simulink model "hdlFrame_LineBufferReuse_MLFB"  (R2025a)
settings: Solver=VariableStepAuto  StartTime=0.0  StopTime=1  RelTol=1e-3
libraries: visionsources x1
settings Model: Creator=navan  LastModifiedBy=kkintali
settings SolverCC: MaxZcPerStep=1.0
settings OptimizationCC: ReuseModelBlockBuffer=off
settings DebuggingCC: UnconnectedInputMsg=warning  UnconnectedOutputMsg=warning  UnconnectedLineMsg=warning
settings ModelReferenceCC: EnableRefExpFcnMdlSchedulingChecks=on
settings SFSimCC: SimDynamicStringBufferSize=Inherit from code generation settings
settings RTWCC: GPUComputeCapability=3.5  DLArmComputeVersion=19.05

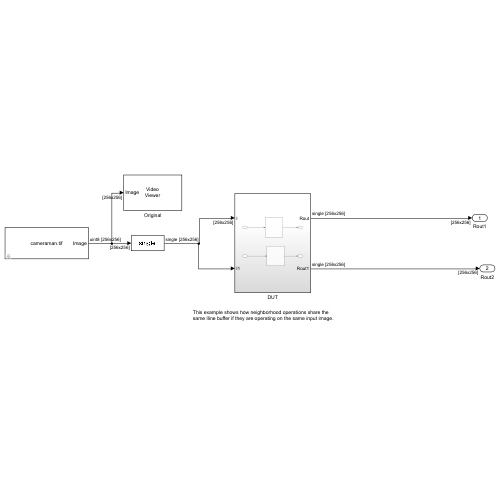
[thumbnail: Simulink's stored preview of the top-level diagram]
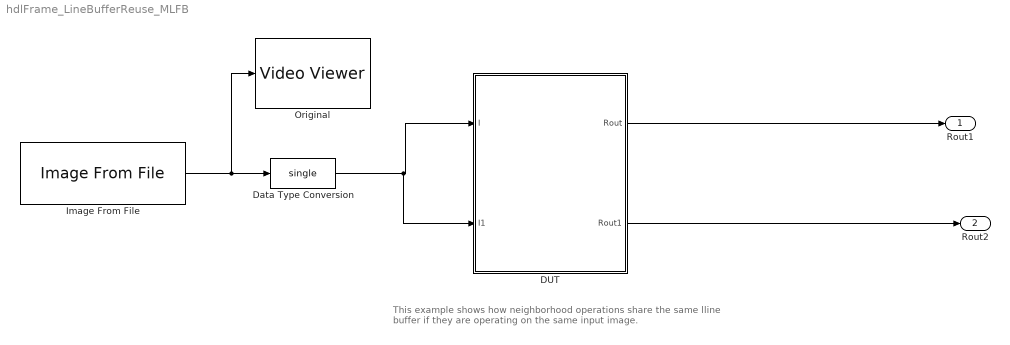
== system hdlFrame_LineBufferReuse_MLFB ==
  note: This example shows how neighborhood operations share the same lline buffer if they are operating on the same input image.
  DUT : Subsystem
  Data Type Conversion : DataTypeConversion  OutDataTypeStr=single  SaturateOnIntegerOverflow=off  RndMeth=Floor
  Image From File : visionsources/Image From File  Tag=vipblks_nd  FileName=cameraman.tif  Ts=1  imagePorts=One multidimensional signal  OutPortLabels=R|G|B  ImageDataType=uint8  sdImageDataType=uint(8)  Signed=on  WordLength=16  FractionLengthMode=User-defined  FractionLength=15
  Original : VideoViewer  FigPos=[1 1438 1396 174]
  Rout1 : Outport
  Rout2 : Outport  Port=2
  wires:
  Data Type Conversion/1 -> DUT/2(I1), DUT/1(I)
  Image From File/1 -> Data Type Conversion/1, Original/1
  DUT/1(Rout) -> Rout1/1
  DUT/2(Rout1) -> Rout2/1

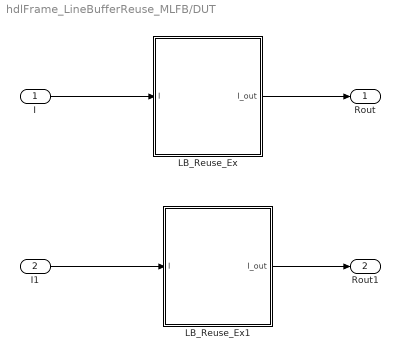
== system hdlFrame_LineBufferReuse_MLFB/DUT ==
  I : Inport
  I1 : Inport  Port=2
  LB_Reuse_Ex : MATLAB Function  TreatAsAtomicUnit=on
  LB_Reuse_Ex1 : MATLAB Function  TreatAsAtomicUnit=on
  Rout : Outport
  Rout1 : Outport  Port=2
  wires:
  I/1 -> LB_Reuse_Ex/1(I)
  LB_Reuse_Ex/1(I_out) -> Rout/1
  LB_Reuse_Ex1/1(I_out) -> Rout1/1
  I1/1 -> LB_Reuse_Ex1/1(I)

== matlab function hdlFrame_LineBufferReuse_MLFB/DUT/LB_Reuse_Ex1 ==
  data: I input; I_out output
function I_out = image_blur(I)
% This example shows both the neighborhood operations below share the same
% line buffer as they are operating on the same image even if the
% neighborhood sizes are different

I_out1 = hdl.npufun(@blur1, [3 3], I);
I_out2 = hdl.npufun(@blur2, [5 5], I);

I_out = I_out1 + I_out2;

end

function y = blur1(N)

y = sum(N(:),'native')/9;

end


function y = blur2(N)

y = sum(N(:),'native')/3;

end

== matlab function hdlFrame_LineBufferReuse_MLFB/DUT/LB_Reuse_Ex ==
  data: I input; I_out output
function I_out = image_blur(I)
% This example shows both the neighborhood operations below share the same
% line buffer as they are operating on the same image.

I_out1 = hdl.npufun(@blur1, [3 3], I);
I_out2 = hdl.npufun(@blur2, [3 3], I);

I_out = I_out1 + I_out2;

end

function y = blur1(N)

y = sum(N(:),'native')/9;

end


function y = blur2(N)

y = sum(N(:),'native')/3;

end
